simulink model "Lab1_placeholder"  (R2025b)
settings: Solver=VariableStepAuto  StartTime=0.0  StopTime=10.0  RelTol=1e-3
values from neighbouring files (symbols this model uses):
  a1 = pi * r1^2    (= 3.14159265359)    [main.m]
  c1 = 1    [main.m]
  h10 = 0.5    [main.m]
settings Model: Creator=adiko  LastModifiedBy=Matadoo

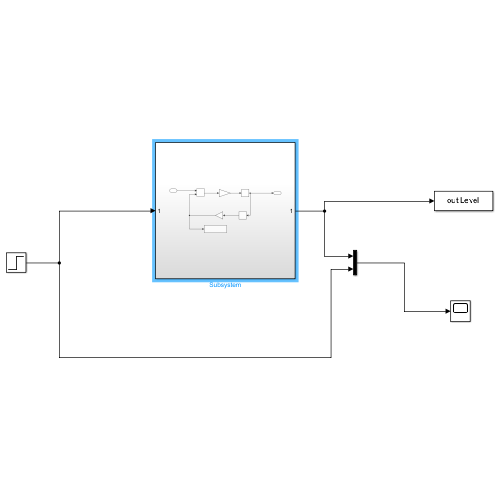
[thumbnail: Simulink's stored preview of the top-level diagram]
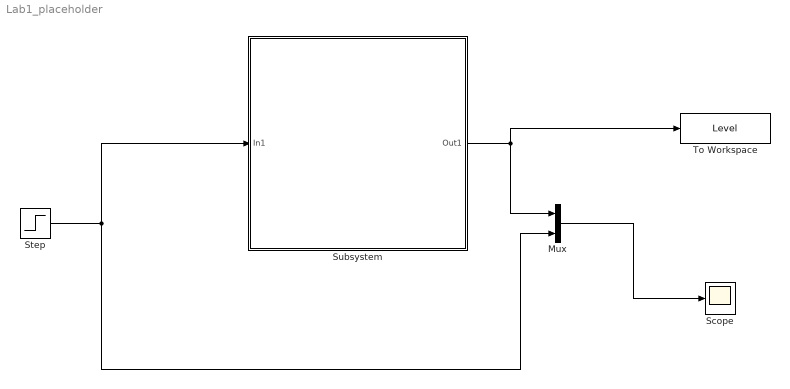
== system Lab1_placeholder ==
  Mux : Mux  Inputs=2
  Scope : Scope
      settings: ActiveDisplayYMinimum=-1  ActiveDisplayYMaximum=1
  Step : Step  Time=0  SampleTime=0
  Subsystem : Subsystem
  To Workspace : ToWorkspace  VariableName=Level  SaveFormat=Timeseries  SampleTime=-1
  wires:
  Mux/1 -> Scope/1
  Step/1 -> Mux/2, Subsystem/1(In1)
  Subsystem/1(Out1) -> Mux/1, To Workspace/1

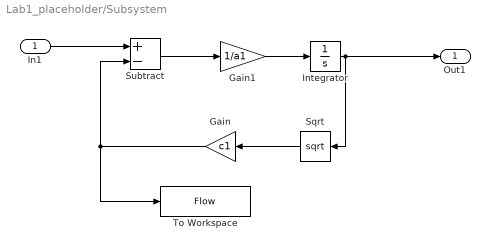
== system Lab1_placeholder/Subsystem ==
  In1 : Inport
  Gain : Gain  Gain=c1
  Gain1 : Gain  Gain=1/a1
  Integrator : Integrator  InitialCondition=h10
  Sqrt : Sqrt
  Subtract : Sum  Inputs=+-
  To Workspace : ToWorkspace  VariableName=Flow  SaveFormat=Timeseries  SampleTime=-1
  Out1 : Outport
  wires:
  In1/1 -> Subtract/1
  Subtract/1 -> Gain1/1
  Gain1/1 -> Integrator/1
  Integrator/1 -> Out1/1, Sqrt/1
  Sqrt/1 -> Gain/1
  Gain/1 -> Subtract/2, To Workspace/1
